simulink model "Task 2 – Battery Modeling"  (R2025b)
settings: Solver=ode23tb  StartTime=0.0  StopTime=35  RelTol=5e-3
model workspace (MAT data in the model file):
  Eng : object (value not decoded)
  Nmtr = 18.5
  SteerLim = 60
  TrackPoints = [-15 -12 -9 -6 -3 5.58745102111e-16 2.81978007367 5.36354042717 7.38228007367 8.67839071119 9.125 8.67839071119 ... (270 elements, 90x3)]
  Trans : object (value not decoded)
  Ts = 0.02
  VEH : object (value not decoded)
symbols that are objects in the model workspace (value not decoded): Eng, Trans, VEH
undefined symbols (not defined in the file or in its folder): BdyFrm, InertFrm
libraries: autolibsharedcoupling x11, simulink x9, sim3dlib x7, autolibutils x5, autolibshareddiff x5, sim3dautolib x3, vehdynlibtirecommon x3, sharedtransform x3, vehdynlibdriver x2, vehdynlibviscommon x2, vehdynlibtire x1, autolibmappedmotor x1
(part 4 of 4)

== system Task 2 – Battery Modeling/Visualization/3D Visualization/Enabled/3D Visualization/Ground Following/Path/Enabled ==
  VehFdbk : Inport
  Bus Selector : BusSelector  OutputSignals=VehFdbk.BdyFrm.Cg.Acc.ax,VehFdbk.BdyFrm.Cg.Acc.ay
  Constant5 : Constant
  Constant6 : Constant  Value=0
  Hypot : Math  Operator=hypot
  Saturation : Saturate  UpperLimit=1  LowerLimit=0  ZeroCross=off
  Simulation 3D Actor : sim3dlib/Simulation 3D Actor  ActorName=GrndVehPath  ParentName=Scene Origin  Operation=Create at setup  InitScriptText=|  SampleTime=Ts*5  Translation=[0 0 0]  Rotation=[0 0 0]  Scale=[1 1 1]  InputsText=PathMarker.Color  aMode=5  ActorTag=GrndVehPath  ActorType=Sim3dActor  ID=C
      | path1 = sim3d.graphics.PathMarker("ActorName", "PathMarker", ControlActorName="SimulinkVehicle3");
      | path1.MarkersSize = ones(1,3)*0.25;
      | path1.Color = [0 0 1];
      | World.add(path1,Actor);
  Sum1 : Sum  Inputs=|++
  Terminator4 : Terminator
  Unary Minus : UnaryMinus
  Vector Concatenate : Concatenate  NumInputs=3  Mode=Multidimensional array  ConcatenateDimension=2
  wires:
  Hypot/1 -> Saturation/1
  Saturation/1 -> Unary Minus/1, Vector Concatenate/1
  Constant5/1 -> Sum1/2
  Simulation 3D Actor/1 -> Terminator4/1
  Sum1/1 -> Vector Concatenate/3
  Unary Minus/1 -> Sum1/1
  Constant6/1 -> Vector Concatenate/2
  VehFdbk/1 -> Bus Selector/1
  Bus Selector/2 -> Hypot/2  "<ay>"
  Bus Selector/1 -> Hypot/1  "<ax>"
  Vector Concatenate/1 -> Simulation 3D Actor/1

== system Task 2 – Battery Modeling/Visualization/3D Visualization/Enabled/3D Visualization/Physical Vehicle/Annotations/Disabled ==

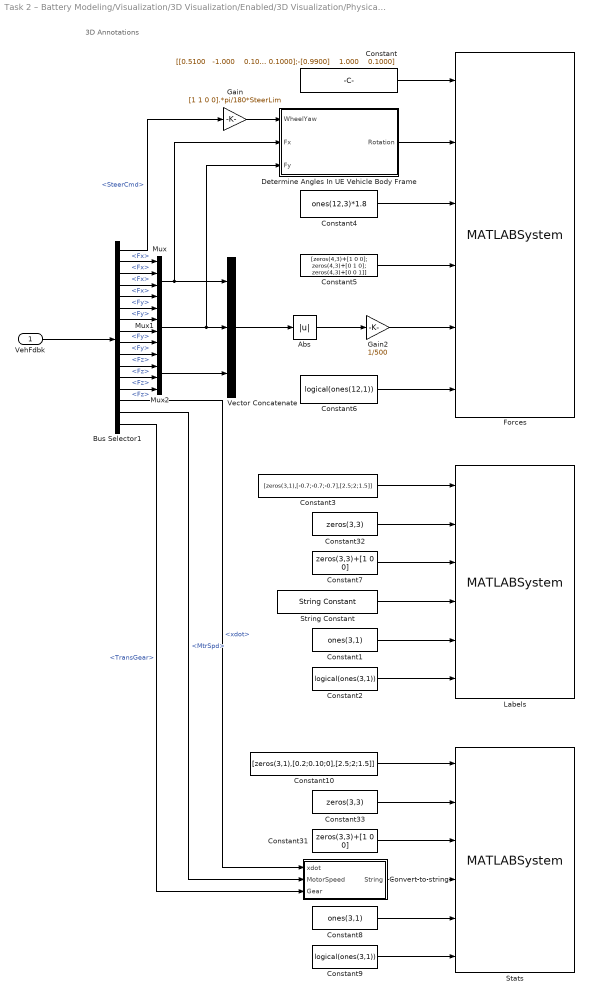
== system Task 2 – Battery Modeling/Visualization/3D Visualization/Enabled/3D Visualization/Physical Vehicle/Annotations/Enabled ==
  note: 3D Annotations
  VehFdbk : Inport
  Abs : Abs  ZeroCross=off  SaturateOnIntegerOverflow=off
  Bus Selector1 : BusSelector  OutputSignals=Driver.SteerCmd,VehFdbk.BdyFrm.Forces.Tires.FrntTires.Lft.Fx,VehFdbk.BdyFrm.Forces.Tires.FrntTires.Rght.Fx,VehFdbk.BdyFrm.Forces.Tires.RearTires.Lft.Fx,VehFdbk.BdyFrm.Forces.Tires.RearTires.Rght.Fx,VehFdbk.BdyFrm.Forces.Tires.FrntTires.Lft.Fy,VehFdbk.BdyFrm.Forces.Tires.FrntTires.Rght.Fy,VehFdbk.BdyFrm.Forces.Tires.RearTires.Lft.Fy,VehFdbk.BdyFrm.Forces.Tires.RearTires.Rght.Fy,VehFdbk.BdyFrm.Forces.Tires.FrntTires.Lft.Fz,VehFdbk.BdyFrm.Forces.Tires.FrntTires.Rght.Fz,VehFdbk.BdyFrm.Forces.Tires.RearTires.Lft.Fz,VehFdbk.BdyFrm.Forces.Tires.RearTires.Rght.Fz,VehFdbk.BdyFrm.Cg.Vel.xdot,VehFdbk.Mtr.MtrSpd,VehFdbk.Trans.TransGear
  Constant : Constant  Value="[[0.5100   -1.000    0.1000];[0.5100    1.000    0.1000];[-0.9900   -1.000    0.1000];[-0.9900    1.000    0.1000];[0.5100   -1.000    0.1000];[0.5100    1.000    0.1000];[-0.9900   -1.000    0.1000];[-0.9900    1.000    0.1000];[0.5100   -1.000    0.1000];[0.5100    1.000    0.1000];[-0.9900   -1.000    0.1000];-[0.9900]    1.000    0.1000]"
  Constant1 : Constant  Value=ones(3,1)
  Constant10 : Constant  Value=[zeros(3,1),[0.2;0.10;0],[2.5;2;1.5]]
  Constant2 : Constant  Value=logical(ones(3,1))
  Constant3 : Constant  Value=[zeros(3,1),[-0.7;-0.7;-0.7],[2.5;2;1.5]]
  Constant31 : Constant  Value=zeros(3,3)+[1 0 0]
  Constant32 : Constant  Value=zeros(3,3)
  Constant33 : Constant  Value=zeros(3,3)
  Constant4 : Constant  Value=ones(12,3)*1.8
  Constant5 : Constant  Value=[zeros(4,3)+[1 0 0]; zeros(4,3)+[0 1 0]; zeros(4,3)+[0 0 1]]
  Constant6 : Constant  Value=logical(ones(12,1))
  Constant7 : Constant  Value=zeros(3,3)+[1 0 0]
  Constant8 : Constant  Value=ones(3,1)
  Constant9 : Constant  Value=logical(ones(3,1))
  Convert to string : Subsystem
  Determine Angles In UE Vehicle Body Frame : Subsystem
  Forces : MATLABSystem  Priority=-1  System=Simulation3DAnnotation  InitialPos="[[0.5100   -1.000    0.1000];[0.5100    1.000    0.1000];[-0.9900   -1.000    0.1000];[-0.9900    1.000    0.1000];[0.5100   -1.000    0.1000];[0.5100    1.000    0.1000];[-0.9900   -1.000    0.1000];[-0.9900    1.000    0.1000];[0.5100   -1.000    0.1000];[0.5100    1.000    0.1000];[-0.9900   -1.000    0.1000];-[0.9900]    1.000    0.1000]"  InitialRot=[zeros(4,3);[zeros(4,3)+[0 0 pi/2]];[zeros(4,3)+[0 pi/2 0]]]  InitialScale=zeros(12,3)  ActorTag=AnnotationActor1  ParentActor=SimulinkVehicle2  Color=[zeros(4,3)+[1 0 0]; zeros(4,3)+[0 1 0]; zeros(4,3)+[0 0 1]]  Length=zeros(12,1)  FontScale=1  IsHidden=logical(zeros(12,1))  SampleTime=Ts
      mask Type: Simulation3DAnnotation
  Gain : Gain  Gain=[1 1 0 0].*pi/180*SteerLim
  Gain2 : Gain  Gain=1/500
  Labels : MATLABSystem  Priority=-1  System=Simulation3DAnnotation  InitialPos=[zeros(3,1),[-0.7;-0.7;-0.7],[2.5;2;1.5]]  InitialRot=zeros(3,3)  InitialScale=zeros(3,3)  ActorTag=AnnotationActor2  ParentActor=SimulinkVehicle2  Color=zeros(3,3)+[1 0 0]  Length=1  String=Velocity\n Engine\n Gear  FontScale=ones(3,1)  IsHidden=logical(ones(3,1))  SampleTime=Ts
      mask Type: Simulation3DAnnotation
  Mux : Mux
  Mux1 : Mux
  Mux2 : Mux
  Stats : MATLABSystem  Priority=-1  System=Simulation3DAnnotation  InitialPos=[zeros(3,1),[0.2;0.1;0.0],[2.5;2;1.5]]  InitialRot=zeros(3,3)  InitialScale=zeros(3,3)  ActorTag=AnnotationActor3  ParentActor=SimulinkVehicle2  Color=zeros(3,3)+[1 0 0]  Length=1  String=00 km/h\n 0000 RPM\n 0  FontScale=ones(3,1)  IsHidden=logical(ones(3,1))  SampleTime=Ts
      mask Type: Simulation3DAnnotation
  String Constant : StringConstant  String="\"Velocity\\n Engine\\n Gear\""
  Vector Concatenate : Concatenate  NumInputs=3
  wires:
  VehFdbk/1 -> Bus Selector1/1
  Determine Angles In UE Vehicle Body Frame/1(Rotation) -> Forces/2
  Mux/1 -> Vector Concatenate/1, Determine Angles In UE Vehicle Body Frame/2(Fx)
  Mux1/1 -> Determine Angles In UE Vehicle Body Frame/3(Fy), Vector Concatenate/2
  Bus Selector1/1 -> Gain/1  "<SteerCmd>"
  Convert to string/1(String) -> Stats/4
  String Constant/1 -> Labels/4
  Constant33/1 -> Stats/2
  Constant31/1 -> Stats/3
  Constant8/1 -> Stats/5
  Constant9/1 -> Stats/6
  Constant32/1 -> Labels/2
  Constant3/1 -> Labels/1
  Constant7/1 -> Labels/3
  Constant1/1 -> Labels/5
  Constant2/1 -> Labels/6
  Constant10/1 -> Stats/1
  Constant/1 -> Forces/1
  Mux2/1 -> Vector Concatenate/3
  Abs/1 -> Gain2/1
  Vector Concatenate/1 -> Abs/1
  Gain2/1 -> Forces/5
  Constant4/1 -> Forces/3
  Constant6/1 -> Forces/6
  Constant5/1 -> Forces/4
  Gain/1 -> Determine Angles In UE Vehicle Body Frame/1(WheelYaw)
  Bus Selector1/2 -> Mux/1  "<Fx>"
  Bus Selector1/3 -> Mux/2  "<Fx>"
  Bus Selector1/4 -> Mux/3  "<Fx>"
  Bus Selector1/5 -> Mux/4  "<Fx>"
  Bus Selector1/6 -> Mux1/1  "<Fy>"
  Bus Selector1/7 -> Mux1/2  "<Fy>"
  Bus Selector1/8 -> Mux1/3  "<Fy>"
  Bus Selector1/9 -> Mux1/4  "<Fy>"
  Bus Selector1/10 -> Mux2/1  "<Fz>"
  Bus Selector1/11 -> Mux2/2  "<Fz>"
  Bus Selector1/12 -> Mux2/3  "<Fz>"
  Bus Selector1/13 -> Mux2/4  "<Fz>"
  Bus Selector1/14 -> Convert to string/1(xdot)  "<xdot>"
  Bus Selector1/15 -> Convert to string/2(MotorSpeed)  "<MtrSpd>"
  Bus Selector1/16 -> Convert to string/3(Gear)  "<TransGear>"

== system Task 2 – Battery Modeling/Visualization/3D Visualization/Enabled/3D Visualization/Physical Vehicle/Path/Disabled ==

== system Task 2 – Battery Modeling/Visualization/3D Visualization/Enabled/3D Visualization/Physical Vehicle/Path/Enabled ==
  VehFdbk : Inport
  Bus Selector : BusSelector  OutputSignals=VehFdbk.BdyFrm.Cg.Acc.ax,VehFdbk.BdyFrm.Cg.Acc.ay
  Constant5 : Constant
  Constant6 : Constant  Value=0
  Hypot : Math  Operator=hypot
  Saturation : Saturate  UpperLimit=1  LowerLimit=0  ZeroCross=off
  Simulation 3D Actor : sim3dlib/Simulation 3D Actor  ActorName=GamePhysVehPath  ParentName=Scene Origin  Operation=Create at setup  InitScriptText=|  SampleTime=Ts*5  Translation=[0 0 0]  Rotation=[0 0 0]  Scale=[1 1 1]  InputsText=PathMarker.Color  aMode=5  ActorTag=GamePhysVehPath  ActorType=Sim3dActor  ID=C
      | path1 = sim3d.graphics.PathMarker("ActorName", "PathMarker", ControlActorName="SimulinkVehicle2");
      | path1.MarkersSize = ones(1,3)*0.25;
      | path1.Color = [0 0 1];
      | World.add(path1,Actor);
  Sum1 : Sum  Inputs=|++
  Terminator4 : Terminator
  Unary Minus : UnaryMinus
  Vector Concatenate : Concatenate  NumInputs=3  Mode=Multidimensional array  ConcatenateDimension=2
  wires:
  Hypot/1 -> Saturation/1
  Saturation/1 -> Unary Minus/1, Vector Concatenate/1
  Constant5/1 -> Sum1/2
  Simulation 3D Actor/1 -> Terminator4/1
  Sum1/1 -> Vector Concatenate/3
  Unary Minus/1 -> Sum1/1
  Constant6/1 -> Vector Concatenate/2
  VehFdbk/1 -> Bus Selector/1
  Bus Selector/2 -> Hypot/2  "<ay>"
  Bus Selector/1 -> Hypot/1  "<ax>"
  Vector Concatenate/1 -> Simulation 3D Actor/1

== system Task 2 – Battery Modeling/Visualization/3D Visualization/Enabled/3D Visualization/Simulation 3D Vehicle/Annotations/Disabled ==

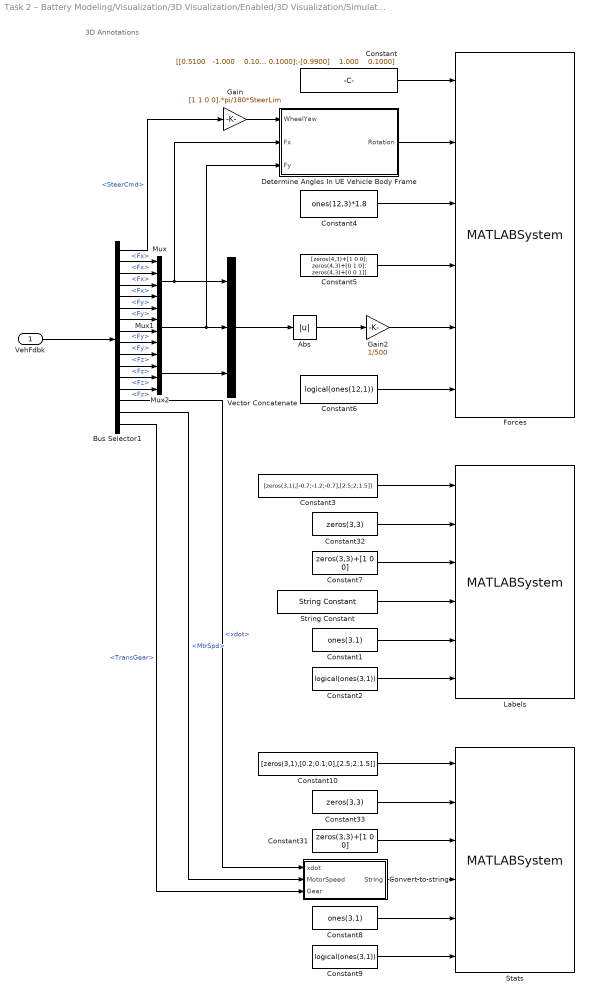
== system Task 2 – Battery Modeling/Visualization/3D Visualization/Enabled/3D Visualization/Simulation 3D Vehicle/Annotations/Enabled ==
  note: 3D Annotations
  VehFdbk : Inport
  Abs : Abs  ZeroCross=off  SaturateOnIntegerOverflow=off
  Bus Selector1 : BusSelector  OutputSignals=Driver.SteerCmd,VehFdbk.BdyFrm.Forces.Tires.FrntTires.Lft.Fx,VehFdbk.BdyFrm.Forces.Tires.FrntTires.Rght.Fx,VehFdbk.BdyFrm.Forces.Tires.RearTires.Lft.Fx,VehFdbk.BdyFrm.Forces.Tires.RearTires.Rght.Fx,VehFdbk.BdyFrm.Forces.Tires.FrntTires.Lft.Fy,VehFdbk.BdyFrm.Forces.Tires.FrntTires.Rght.Fy,VehFdbk.BdyFrm.Forces.Tires.RearTires.Lft.Fy,VehFdbk.BdyFrm.Forces.Tires.RearTires.Rght.Fy,VehFdbk.BdyFrm.Forces.Tires.FrntTires.Lft.Fz,VehFdbk.BdyFrm.Forces.Tires.FrntTires.Rght.Fz,VehFdbk.BdyFrm.Forces.Tires.RearTires.Lft.Fz,VehFdbk.BdyFrm.Forces.Tires.RearTires.Rght.Fz,VehFdbk.BdyFrm.Cg.Vel.xdot,VehFdbk.Mtr.MtrSpd,VehFdbk.Trans.TransGear
  Constant : Constant  Value="[[0.5100   -1.000    0.1000];[0.5100    1.000    0.1000];[-0.9900   -1.000    0.1000];[-0.9900    1.000    0.1000];[0.5100   -1.000    0.1000];[0.5100    1.000    0.1000];[-0.9900   -1.000    0.1000];[-0.9900    1.000    0.1000];[0.5100   -1.000    0.1000];[0.5100    1.000    0.1000];[-0.9900   -1.000    0.1000];-[0.9900]    1.000    0.1000]"
  Constant1 : Constant  Value=ones(3,1)
  Constant10 : Constant  Value=[zeros(3,1),[0.2;0.1;0],[2.5;2;1.5]]
  Constant2 : Constant  Value=logical(ones(3,1))
  Constant3 : Constant  Value=[zeros(3,1),[-0.7;-1.2;-0.7],[2.5;2;1.5]]
  Constant31 : Constant  Value=zeros(3,3)+[1 0 0]
  Constant32 : Constant  Value=zeros(3,3)
  Constant33 : Constant  Value=zeros(3,3)
  Constant4 : Constant  Value=ones(12,3)*1.8
  Constant5 : Constant  Value=[zeros(4,3)+[1 0 0]; zeros(4,3)+[0 1 0]; zeros(4,3)+[0 0 1]]
  Constant6 : Constant  Value=logical(ones(12,1))
  Constant7 : Constant  Value=zeros(3,3)+[1 0 0]
  Constant8 : Constant  Value=ones(3,1)
  Constant9 : Constant  Value=logical(ones(3,1))
  Convert to string : Subsystem
  Determine Angles In UE Vehicle Body Frame : Subsystem
  Forces : MATLABSystem  Priority=-1  System=Simulation3DAnnotation  InitialPos="[[0.5100   -1.000    0.1000];[0.5100    1.000    0.1000];[-0.9900   -1.000    0.1000];[-0.9900    1.000    0.1000];[0.5100   -1.000    0.1000];[0.5100    1.000    0.1000];[-0.9900   -1.000    0.1000];[-0.9900    1.000    0.1000];[0.5100   -1.000    0.1000];[0.5100    1.000    0.1000];[-0.9900   -1.000    0.1000];-[0.9900]    1.000    0.1000]"  InitialRot=[zeros(4,3);[zeros(4,3)+[0 0 pi/2]];[zeros(4,3)+[0 pi/2 0]]]  InitialScale=zeros(12,3)  ActorTag=AnnotationActor1  ParentActor=SimulinkVehicle1  Color=[zeros(4,3)+[1 0 0]; zeros(4,3)+[0 1 0]; zeros(4,3)+[0 0 1]]  Length=zeros(12,1)  FontScale=1  IsHidden=logical(zeros(12,1))  SampleTime=Ts
      mask Type: Simulation3DAnnotation
  Gain : Gain  Gain=[1 1 0 0].*pi/180*SteerLim
  Gain2 : Gain  Gain=1/500
  Labels : MATLABSystem  Priority=-1  System=Simulation3DAnnotation  InitialPos=[zeros(3,1),[-0.7;-0.7;-0.7],[2.5;2;1.5]]  InitialRot=zeros(3,3)  InitialScale=zeros(3,3)  ActorTag=AnnotationActor2  ParentActor=SimulinkVehicle1  Color=zeros(3,3)+[1 0 0]  Length=1  String=Velocity\n Motor (max)\n Gear  FontScale=ones(3,1)  IsHidden=logical(ones(3,1))  SampleTime=Ts
      mask Type: Simulation3DAnnotation
  Mux : Mux
  Mux1 : Mux
  Mux2 : Mux
  Stats : MATLABSystem  Priority=-1  System=Simulation3DAnnotation  InitialPos=[zeros(3,1),[0.2;0.1;0],[2.5;2;1.5]]  InitialRot=zeros(3,3)  InitialScale=zeros(3,3)  ActorTag=AnnotationActor3  ParentActor=SimulinkVehicle1  Color=zeros(3,3)+[1 0 0]  Length=1  String=00 km/h\n 0000 RPM\n 0  FontScale=ones(3,1)  IsHidden=logical(ones(3,1))  SampleTime=Ts
      mask Type: Simulation3DAnnotation
  String Constant : StringConstant  String="\"Velocity\\n Max Motor \\n Gear\""
  Vector Concatenate : Concatenate  NumInputs=3
  wires:
  VehFdbk/1 -> Bus Selector1/1
  Determine Angles In UE Vehicle Body Frame/1(Rotation) -> Forces/2
  Mux/1 -> Vector Concatenate/1, Determine Angles In UE Vehicle Body Frame/2(Fx)
  Mux1/1 -> Determine Angles In UE Vehicle Body Frame/3(Fy), Vector Concatenate/2
  Bus Selector1/1 -> Gain/1  "<SteerCmd>"
  Convert to string/1(String) -> Stats/4
  String Constant/1 -> Labels/4
  Constant33/1 -> Stats/2
  Constant31/1 -> Stats/3
  Constant8/1 -> Stats/5
  Constant9/1 -> Stats/6
  Constant32/1 -> Labels/2
  Constant3/1 -> Labels/1
  Constant7/1 -> Labels/3
  Constant1/1 -> Labels/5
  Constant2/1 -> Labels/6
  Constant10/1 -> Stats/1
  Constant/1 -> Forces/1
  Mux2/1 -> Vector Concatenate/3
  Abs/1 -> Gain2/1
  Vector Concatenate/1 -> Abs/1
  Gain2/1 -> Forces/5
  Constant4/1 -> Forces/3
  Constant6/1 -> Forces/6
  Constant5/1 -> Forces/4
  Gain/1 -> Determine Angles In UE Vehicle Body Frame/1(WheelYaw)
  Bus Selector1/2 -> Mux/1  "<Fx>"
  Bus Selector1/3 -> Mux/2  "<Fx>"
  Bus Selector1/4 -> Mux/3  "<Fx>"
  Bus Selector1/5 -> Mux/4  "<Fx>"
  Bus Selector1/6 -> Mux1/1  "<Fy>"
  Bus Selector1/7 -> Mux1/2  "<Fy>"
  Bus Selector1/8 -> Mux1/3  "<Fy>"
  Bus Selector1/9 -> Mux1/4  "<Fy>"
  Bus Selector1/10 -> Mux2/1  "<Fz>"
  Bus Selector1/11 -> Mux2/2  "<Fz>"
  Bus Selector1/12 -> Mux2/3  "<Fz>"
  Bus Selector1/13 -> Mux2/4  "<Fz>"
  Bus Selector1/14 -> Convert to string/1(xdot)  "<xdot>"
  Bus Selector1/15 -> Convert to string/2(MotorSpeed)  "<MtrSpd>"
  Bus Selector1/16 -> Convert to string/3(Gear)  "<TransGear>"

== system Task 2 – Battery Modeling/Visualization/3D Visualization/Enabled/3D Visualization/Simulation 3D Vehicle/Path/Disabled ==

== system Task 2 – Battery Modeling/Visualization/3D Visualization/Enabled/3D Visualization/Simulation 3D Vehicle/Path/Enabled ==
  VehFdbk : Inport
  Bus Selector : BusSelector  OutputSignals=VehFdbk.BdyFrm.Cg.Acc.ax,VehFdbk.BdyFrm.Cg.Acc.ay
  Constant5 : Constant
  Constant6 : Constant  Value=0
  Hypot : Math  Operator=hypot
  Saturation : Saturate  UpperLimit=1  LowerLimit=0  ZeroCross=off
  Simulation 3D Actor : sim3dlib/Simulation 3D Actor  Priority=10  ActorName=SimulinkPhysVehPath  ParentName=Scene Origin  Operation=Create at setup  InitScriptText=|  SampleTime=Ts*5  Translation=[0 0 0]  Rotation=[0 0 0]  Scale=[1 1 1]  InputsText=PathMarker.Color  aMode=5  ActorTag=SimulinkPhysVehPath  ActorType=Sim3dActor  ID=C
      | path1 = sim3d.graphics.PathMarker("ActorName", "PathMarker", ControlActorName="SimulinkVehicle1");
      | path1.MarkersSize = ones(1,3)*0.25;
      | path1.Color = [0 0 1];
      | World.add(path1,Actor);
  Sum1 : Sum  Inputs=|++
  Terminator4 : Terminator
  Unary Minus : UnaryMinus
  Vector Concatenate : Concatenate  NumInputs=3  Mode=Multidimensional array  ConcatenateDimension=2
  wires:
  Hypot/1 -> Saturation/1
  Saturation/1 -> Unary Minus/1, Vector Concatenate/1
  Constant5/1 -> Sum1/2
  Simulation 3D Actor/1 -> Terminator4/1
  Sum1/1 -> Vector Concatenate/3
  Unary Minus/1 -> Sum1/1
  Constant6/1 -> Vector Concatenate/2
  VehFdbk/1 -> Bus Selector/1
  Bus Selector/2 -> Hypot/2  "<ay>"
  Bus Selector/1 -> Hypot/1  "<ax>"
  Vector Concatenate/1 -> Simulation 3D Actor/1

== system Task 2 – Battery Modeling/Visualization/3D Visualization/Enabled/3D Visualization/Simulation 3D Vehicle/Scale/PartConcatenation ==
  BodyX : Inport
  BodyY : Inport  Port=2
  BodyZ : Inport  Port=3
  WheelFrontLeftX : Inport  Port=4
  WheelFrontLeftY : Inport  Port=5
  WheelFrontLeftZ : Inport  Port=6
  WheelFrontRightX : Inport  Port=7
  WheelFrontRightY : Inport  Port=8
  WheelFrontRightZ : Inport  Port=9
  WheelRearLeftX : Inport  Port=10
  WheelRearLeftY : Inport  Port=11
  WheelRearLeftZ : Inport  Port=12
  WheelRearRightX : Inport  Port=13
  WheelRearRightY : Inport  Port=14
  WheelRearRightZ : Inport  Port=15
  AllParts : Concatenate  NumInputs=5  Mode=Multidimensional array
  Body : Concatenate  NumInputs=3  Mode=Multidimensional array  ConcatenateDimension=2
  WheelFrontLeft : Concatenate  NumInputs=3  Mode=Multidimensional array  ConcatenateDimension=2
  WheelFrontRight : Concatenate  NumInputs=3  Mode=Multidimensional array  ConcatenateDimension=2
  WheelRearLeft : Concatenate  NumInputs=3  Mode=Multidimensional array  ConcatenateDimension=2
  WheelRearRight : Concatenate  NumInputs=3  Mode=Multidimensional array  ConcatenateDimension=2
  ConcatOut : Outport  VectorParamsAs1DForOutWhenUnconnected=off
  wires:
  BodyX/1 -> Body/1
  BodyZ/1 -> Body/3
  WheelFrontLeftX/1 -> WheelFrontLeft/1
  WheelFrontLeftZ/1 -> WheelFrontLeft/3
  WheelFrontLeftY/1 -> WheelFrontLeft/2
  BodyY/1 -> Body/2
  WheelFrontLeft/1 -> AllParts/2
  WheelRearRightX/1 -> WheelRearRight/1
  Body/1 -> AllParts/1
  WheelRearLeft/1 -> AllParts/4
  WheelFrontRight/1 -> AllParts/3
  WheelRearRightZ/1 -> WheelRearRight/3
  WheelFrontRightY/1 -> WheelFrontRight/2
  WheelFrontRightX/1 -> WheelFrontRight/1
  WheelRearRightY/1 -> WheelRearRight/2
  WheelRearLeftZ/1 -> WheelRearLeft/3
  AllParts/1 -> ConcatOut/1
  WheelRearLeftY/1 -> WheelRearLeft/2
  WheelRearRight/1 -> AllParts/5
  WheelRearLeftX/1 -> WheelRearLeft/1
  WheelFrontRightZ/1 -> WheelFrontRight/3

== system Task 2 – Battery Modeling/Visualization/3D Visualization/Enabled/3D Visualization/Ground Following/Annotations/Enabled/Convert to string ==
  xdot : Inport
  MotorSpeed : Inport  Port=2
  Gear : Inport  Port=3
  Round : Rounding  Operator=round
  Round1 : Rounding  Operator=round
  Signal Specification : SignalSpecification  Unit=rpm
  Signal Specification1 : SignalSpecification  Unit=km/h
  String Concatenate1 : StringConcatenate  Inputs=3
  String Concatenate2 : StringConcatenate
  String Concatenate3 : StringConcatenate
  String Constant3 : StringConstant  String="\" km/h\\n\""
  String Constant4 : StringConstant  String="\" RPM\\n\""
  To String1 : ToString
  To String2 : ToString
  To String3 : ToString
  Unit Conversion : UnitConversion
  Unit Conversion1 : UnitConversion
  String : Outport
  wires:
  MotorSpeed/1 -> Unit Conversion/1
  Signal Specification/1 -> Round1/1
  String Constant4/1 -> String Concatenate3/2
  Signal Specification1/1 -> Round/1
  String Concatenate2/1 -> String Concatenate1/1
  To String2/1 -> String Concatenate2/1
  String Constant3/1 -> String Concatenate2/2
  To String1/1 -> String Concatenate1/3
  String Concatenate3/1 -> String Concatenate1/2
  To String3/1 -> String Concatenate3/1
  Round/1 -> To String2/1
  Round1/1 -> To String3/1
  String Concatenate1/1 -> String/1
  Gear/1 -> To String1/1
  Unit Conversion/1 -> Signal Specification/1
  Unit Conversion1/1 -> Signal Specification1/1
  xdot/1 -> Unit Conversion1/1

== system Task 2 – Battery Modeling/Visualization/3D Visualization/Enabled/3D Visualization/Ground Following/Annotations/Enabled/Determine Angles In UE Vehicle Body Frame ==
  WheelYaw : Inport
  Fx : Inport  Port=2
  Fy : Inport  Port=3
  Add : Sum
  Add1 : Sum
  Constant1 : Constant  Value=0
  Constant11 : Constant  Value=[zeros(4,1)]
  Constant12 : Constant  Value=[zeros(4,1); ones(4,1).*pi/2]
  Constant2 : Constant  Value=pi
  Constant3 : Constant  Value=[zeros(8,2)]
  Constant4 : Constant  Value=[zeros(12,2)]
  Constant6 : Constant  Value=repmat([0 pi/2 0],[4,1])
  Matrix Concatenate : Concatenate  Mode=Multidimensional array
  Matrix Concatenate1 : Concatenate  Mode=Multidimensional array  ConcatenateDimension=2
  Matrix Concatenate2 : Concatenate  Mode=Multidimensional array
  Matrix Concatenate3 : Concatenate  NumInputs=3  Mode=Multidimensional array
  Matrix Concatenate4 : Concatenate  Mode=Multidimensional array  ConcatenateDimension=2
  Switch8 : Switch  ZeroCross=off  SaturateOnIntegerOverflow=off  InputSameDT=off
  Rotation : Outport
  wires:
  Constant2/1 -> Switch8/1
  Matrix Concatenate2/1 -> Switch8/2
  Constant1/1 -> Switch8/3
  Constant3/1 -> Matrix Concatenate1/1
  Matrix Concatenate1/1 -> Matrix Concatenate/1
  Switch8/1 -> Add/1
  Constant6/1 -> Matrix Concatenate/2
  Fx/1 -> Matrix Concatenate2/1
  Fy/1 -> Matrix Concatenate2/2
  Add/1 -> Matrix Concatenate1/2
  Constant12/1 -> Add/2
  Constant11/1 -> Matrix Concatenate3/3
  WheelYaw/1 -> Matrix Concatenate3/1, Matrix Concatenate3/2
  Constant4/1 -> Matrix Concatenate4/1
  Matrix Concatenate3/1 -> Matrix Concatenate4/2
  Matrix Concatenate4/1 -> Add1/2
  Matrix Concatenate/1 -> Add1/1
  Add1/1 -> Rotation/1

== system Task 2 – Battery Modeling/Visualization/3D Visualization/Enabled/3D Visualization/Physical Vehicle/Annotations/Enabled/Convert to string ==
  xdot : Inport
  MotorSpeed : Inport  Port=2
  Gear : Inport  Port=3
  Round : Rounding  Operator=round
  Round1 : Rounding  Operator=round
  Signal Specification : SignalSpecification  Unit=rpm
  Signal Specification1 : SignalSpecification  Unit=km/h
  String Concatenate1 : StringConcatenate  Inputs=3
  String Concatenate2 : StringConcatenate
  String Concatenate3 : StringConcatenate
  String Constant3 : StringConstant  String="\" km/h\\n\""
  String Constant4 : StringConstant  String="\" RPM\\n\""
  To String1 : ToString
  To String2 : ToString
  To String3 : ToString
  Unit Conversion : UnitConversion
  Unit Conversion1 : UnitConversion
  String : Outport
  wires:
  MotorSpeed/1 -> Unit Conversion/1
  Signal Specification/1 -> Round1/1
  String Constant4/1 -> String Concatenate3/2
  Signal Specification1/1 -> Round/1
  String Concatenate2/1 -> String Concatenate1/1
  To String2/1 -> String Concatenate2/1
  String Constant3/1 -> String Concatenate2/2
  To String1/1 -> String Concatenate1/3
  String Concatenate3/1 -> String Concatenate1/2
  To String3/1 -> String Concatenate3/1
  Round/1 -> To String2/1
  Round1/1 -> To String3/1
  String Concatenate1/1 -> String/1
  Gear/1 -> To String1/1
  Unit Conversion/1 -> Signal Specification/1
  Unit Conversion1/1 -> Signal Specification1/1
  xdot/1 -> Unit Conversion1/1

== system Task 2 – Battery Modeling/Visualization/3D Visualization/Enabled/3D Visualization/Physical Vehicle/Annotations/Enabled/Determine Angles In UE Vehicle Body Frame ==
  WheelYaw : Inport
  Fx : Inport  Port=2
  Fy : Inport  Port=3
  Add : Sum
  Add1 : Sum
  Constant1 : Constant  Value=0
  Constant11 : Constant  Value=[zeros(4,1)]
  Constant12 : Constant  Value=[zeros(4,1); ones(4,1).*pi/2]
  Constant2 : Constant  Value=pi
  Constant3 : Constant  Value=[zeros(8,2)]
  Constant4 : Constant  Value=[zeros(12,2)]
  Constant6 : Constant  Value=repmat([0 pi/2 0],[4,1])
  Matrix Concatenate : Concatenate  Mode=Multidimensional array
  Matrix Concatenate1 : Concatenate  Mode=Multidimensional array  ConcatenateDimension=2
  Matrix Concatenate2 : Concatenate  Mode=Multidimensional array
  Matrix Concatenate3 : Concatenate  NumInputs=3  Mode=Multidimensional array
  Matrix Concatenate4 : Concatenate  Mode=Multidimensional array  ConcatenateDimension=2
  Switch8 : Switch  ZeroCross=off  SaturateOnIntegerOverflow=off  InputSameDT=off
  Rotation : Outport
  wires:
  Constant2/1 -> Switch8/1
  Matrix Concatenate2/1 -> Switch8/2
  Constant1/1 -> Switch8/3
  Constant3/1 -> Matrix Concatenate1/1
  Matrix Concatenate1/1 -> Matrix Concatenate/1
  Switch8/1 -> Add/1
  Constant6/1 -> Matrix Concatenate/2
  Fx/1 -> Matrix Concatenate2/1
  Fy/1 -> Matrix Concatenate2/2
  Add/1 -> Matrix Concatenate1/2
  Constant12/1 -> Add/2
  Constant11/1 -> Matrix Concatenate3/3
  WheelYaw/1 -> Matrix Concatenate3/1, Matrix Concatenate3/2
  Constant4/1 -> Matrix Concatenate4/1
  Matrix Concatenate3/1 -> Matrix Concatenate4/2
  Matrix Concatenate4/1 -> Add1/2
  Matrix Concatenate/1 -> Add1/1
  Add1/1 -> Rotation/1

== system Task 2 – Battery Modeling/Visualization/3D Visualization/Enabled/3D Visualization/Simulation 3D Vehicle/Annotations/Enabled/Convert to string ==
  xdot : Inport
  MotorSpeed : Inport  Port=2
  Gear : Inport  Port=3
  Max : MinMax  Function=max  ZeroCross=off
  Round : Rounding  Operator=round
  Round1 : Rounding  Operator=round
  Signal Specification : SignalSpecification  Unit=rpm
  Signal Specification1 : SignalSpecification  Unit=km/h
  String Concatenate1 : StringConcatenate  Inputs=3
  String Concatenate2 : StringConcatenate
  String Concatenate3 : StringConcatenate
  String Constant3 : StringConstant  String="\" km/h\\n\""
  String Constant4 : StringConstant  String="\" RPM\\n\""
  To String1 : ToString
  To String2 : ToString
  To String3 : ToString
  Unit Conversion : UnitConversion
  Unit Conversion1 : UnitConversion
  String : Outport
  wires:
  MotorSpeed/1 -> Unit Conversion/1
  Signal Specification/1 -> Round1/1
  String Constant4/1 -> String Concatenate3/2
  Signal Specification1/1 -> Round/1
  String Concatenate2/1 -> String Concatenate1/1
  To String2/1 -> String Concatenate2/1
  String Constant3/1 -> String Concatenate2/2
  To String1/1 -> String Concatenate1/3
  String Concatenate3/1 -> String Concatenate1/2
  To String3/1 -> String Concatenate3/1
  Round/1 -> To String2/1
  Round1/1 -> Max/1
  String Concatenate1/1 -> String/1
  Gear/1 -> To String1/1
  Unit Conversion/1 -> Signal Specification/1
  Unit Conversion1/1 -> Signal Specification1/1
  xdot/1 -> Unit Conversion1/1
  Max/1 -> To String3/1

== system Task 2 – Battery Modeling/Visualization/3D Visualization/Enabled/3D Visualization/Simulation 3D Vehicle/Annotations/Enabled/Determine Angles In UE Vehicle Body Frame ==
  WheelYaw : Inport
  Fx : Inport  Port=2
  Fy : Inport  Port=3
  Add : Sum
  Add1 : Sum
  Constant1 : Constant  Value=0
  Constant11 : Constant  Value=[zeros(4,1)]
  Constant12 : Constant  Value=[zeros(4,1); ones(4,1).*pi/2]
  Constant2 : Constant  Value=pi
  Constant3 : Constant  Value=[zeros(8,2)]
  Constant4 : Constant  Value=[zeros(12,2)]
  Constant6 : Constant  Value=repmat([0 pi/2 0],[4,1])
  Matrix Concatenate : Concatenate  Mode=Multidimensional array
  Matrix Concatenate1 : Concatenate  Mode=Multidimensional array  ConcatenateDimension=2
  Matrix Concatenate2 : Concatenate  Mode=Multidimensional array
  Matrix Concatenate3 : Concatenate  NumInputs=3  Mode=Multidimensional array
  Matrix Concatenate4 : Concatenate  Mode=Multidimensional array  ConcatenateDimension=2
  Switch8 : Switch  ZeroCross=off  SaturateOnIntegerOverflow=off  InputSameDT=off
  Rotation : Outport
  wires:
  Constant2/1 -> Switch8/1
  Matrix Concatenate2/1 -> Switch8/2
  Constant1/1 -> Switch8/3
  Constant3/1 -> Matrix Concatenate1/1
  Matrix Concatenate1/1 -> Matrix Concatenate/1
  Switch8/1 -> Add/1
  Constant6/1 -> Matrix Concatenate/2
  Fx/1 -> Matrix Concatenate2/1
  Fy/1 -> Matrix Concatenate2/2
  Add/1 -> Matrix Concatenate1/2
  Constant12/1 -> Add/2
  Constant11/1 -> Matrix Concatenate3/3
  WheelYaw/1 -> Matrix Concatenate3/1, Matrix Concatenate3/2
  Constant4/1 -> Matrix Concatenate4/1
  Matrix Concatenate3/1 -> Matrix Concatenate4/2
  Matrix Concatenate4/1 -> Add1/2
  Matrix Concatenate/1 -> Add1/1
  Add1/1 -> Rotation/1

== matlab function Task 2 – Battery Modeling/Formula Student Vehicle/Simulink Physics - 7DOF/Powertrain & Driveline/Powertrain/4EM Powertrain/Torque Management ==
  data: Acc input; HndWhl input; MtrTrqCmd output; r input
function MtrTrqCmd = trqmngr(Acc, HndWhl, r) %#codegen
% Copyright MathWorks Inc. 2024
Tmax = 5;
rmax = 500*pi/180;
Kr = 15;
MtrTrqCmd = ones(4,1).*Acc;
yawDiff = HndWhl - r./rmax;
MtrTrqCmd = (MtrTrqCmd +[1 -1 1 -1]'.*Kr.*yawDiff).*Tmax; 
maxTinds = abs(MtrTrqCmd)>Tmax;
MtrTrqCmd(maxTinds) = Tmax.*sign(MtrTrqCmd(maxTinds));

== matlab function Task 2 – Battery Modeling/Skidpad Reference/Lap Time Counter ==
  settings: updateMethod=DISCRETE
  data: X input; LapTimes output; Y input; psi input; t input; CurrLapNum output
function [LapTimes, CurrLapNum]  = laptimer(X, Y, psi, t)
% A very simple lap counter. Assumes the start line is at X = 0, along Y
% axis within a specified track width
%
% Copyright 2022 The MathWorks, Inc.
%
%#codegen
coder.allowpcode('plain')
NLaps = 4;
trackWidth = 3.5; 
[LapTimes, CurrLapNum] = vdynlaptimer(X, Y, psi, t,NLaps,trackWidth);
end

== matlab function Task 2 – Battery Modeling/Formula Student Vehicle/Simulink Physics - 7DOF/Powertrain & Driveline/Powertrain/4EM Powertrain/MATLAB Function ==
  data: I input; V_batt output; SOC output
function [V_batt, SOC] = fcn(I)

Q = 2 * 3600;

   % 2Ah battery capacity
R = 0.03;        % internal resistance
dt = 0.01;       % sample time

persistent soc

if isempty(soc)
    soc = 1;     % start at 100% SOC
end

% SOC calculation
soc = soc - (I * dt) / Q;
soc = min(max(soc,0),1);

% Voltage model (range 180–220V)
OCV = 180 + 40*soc;

V_single = OCV - I*R;

% 4 motors need 4 voltages
V_batt = V_single * ones(4,1);

SOC = soc;
